simulink model "TB24_StageA_ModuleFault"  (R2025a)
settings: Solver=FixedStepDiscrete  StartTime=0  StopTime=TB.t_end  FixedStep=TB.dt  RelTol=1e-3
InitFcn:
  | % 모델과 같은 폴더의 초기화 스크립트를 실행해 P(설계 파라미터)와 TB(시험 조건)를 만든다.
  | run(fullfile(fileparts(get_param(bdroot, 'FileName')), 'TB24_init.m'));
values from neighbouring files (symbols this model uses):
  TB = struct()    [TB24_init.m]    (also in run_TB24.m = evalin('base', 'TB'))
libraries: fl_lib x126, nesl_utility x55
(part 2 of 3)

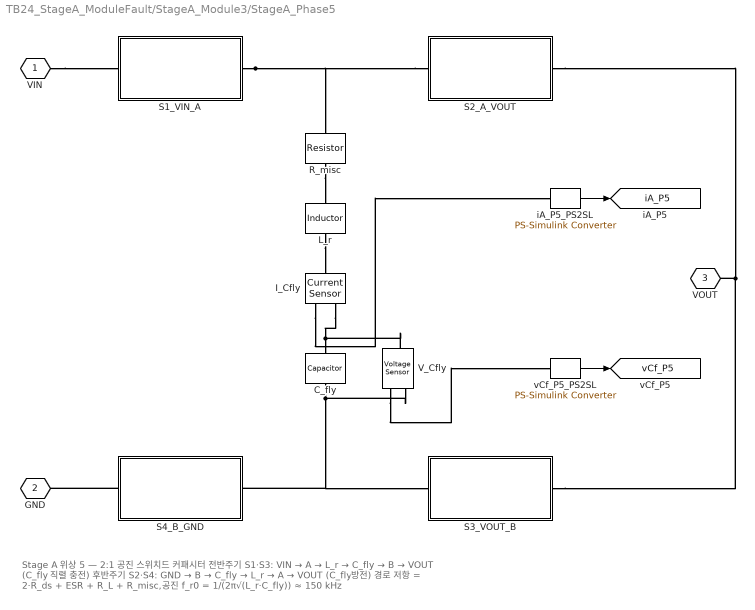
== system TB24_StageA_ModuleFault/StageA_Module3/StageA_Phase5 ==
  note: Stage A 위상 5 — 2:1 공진 스위치드 커패시터
      | 전반주기 S1·S3: VIN → A → L_r → C_fly → B → VOUT (C_fly 직렬 충전)
      | 후반주기 S2·S4: GND → B → C_fly → L_r → A → VOUT (C_fly 방전)
      | 경로 저항 = 2·R_ds + ESR + R_L + R_misc, 공진 f_r0 = 1/(2π√(L_r·C_fly)) ≈ 150 kHz
  C_fly : fl_lib/Electrical/Electrical Elements/Capacitor  c=TB.A.Cfly F  r=TB.A.ESR Ohm  g=0 1/Ohm  i_specify=off  i_priority=None  i=0 A  i_nominal_specify=off  i_nominal_value=1  i_nominal_unit=A  v_specify=off  v_priority=None  v=0 V  v_nominal_specify=off  v_nominal_value=1  v_nominal_unit=V  vc_specify=on  vc_priority=High  vc=TB.vC0_ph(5) V  vc_nominal_specify=off  vc_nominal_value=1  vc_nominal_unit=V
  I_Cfly : fl_lib/Electrical/Electrical Sensors/Current Sensor
  L_r : fl_lib/Electrical/Electrical Elements/Inductor  l=TB.A.Lr H  r=TB.A.RL Ohm  g=1e-9 1/Ohm  i_specify=off  i_priority=None  i=0 A  i_nominal_specify=off  i_nominal_value=1  i_nominal_unit=A  v_specify=off  v_priority=None  v=0 V  v_nominal_specify=off  v_nominal_value=1  v_nominal_unit=V  i_L_specify=on  i_L_priority=High  i_L=0 A  i_L_nominal_specify=off  i_L_nominal_value=1  i_L_nominal_unit=A
  R_misc : fl_lib/Electrical/Electrical Elements/Resistor  R=TB.A.Rmisc Ohm  i_specify=off  i_priority=None  i=0 A  i_nominal_specify=off  i_nominal_value=1  i_nominal_unit=A  v_specify=off  v_priority=None  v=0 V  v_nominal_specify=off  v_nominal_value=1  v_nominal_unit=V
  S1_VIN_A : Subsystem  mask(PRISM-Hub switch cell){Ron=TB.A.Rds, Goff=TB.A.Goff, Vf=TB.A.Vf, Rd=TB.A.Rd, Goffd=TB.A.Goffd}
      mask prompts: Ron "도통 저항 R_on [Ohm]"; Goff "차단 컨덕턴스 G_off [S]"; Vf "다이오드 순방향 전압 Vf [V]"; Rd "다이오드 도통 저항 R_d [Ohm]"; Goffd "다이오드 차단 컨덕턴스 [S]"
      mask help: 전력 반도체 스위치 셀 S1. 게이트 태그 gA_P5_S1.
      settings: AttributesFormatString=gate: gA_P5_S1
      mask Display:
      | plot([0.05 0.35 ],[0.50 0.50 ],[0.35 0.65 ],[0.50 0.74 ],[0.65 0.95 ],[0.50 0.50 ]);
      | plot([0.20 0.20 0.42 ],[0.50 0.20 0.20 ],[0.58 0.80 0.80 ],[0.20 0.20 0.50 ]);
      | plot([0.42 0.58 0.58 0.42 ],[0.20 0.10 0.30 0.20 ],[0.42 0.42 ],[0.10 0.30 ]);
      | text(0.5,0.80,'S1','horizontalAlignment','center','texmode','off');
      | port_label('LConn',1,'D');
      | port_label('RConn',1,'S');
  S2_A_VOUT : Subsystem  mask(PRISM-Hub switch cell){Ron=TB.A.Rds, Goff=TB.A.Goff, Vf=TB.A.Vf, Rd=TB.A.Rd, Goffd=TB.A.Goffd}
      mask prompts: Ron "도통 저항 R_on [Ohm]"; Goff "차단 컨덕턴스 G_off [S]"; Vf "다이오드 순방향 전압 Vf [V]"; Rd "다이오드 도통 저항 R_d [Ohm]"; Goffd "다이오드 차단 컨덕턴스 [S]"
      mask help: 전력 반도체 스위치 셀 S2. 게이트 태그 gA_P5_S2.
      settings: AttributesFormatString=gate: gA_P5_S2
      mask Display:
      | plot([0.05 0.35 ],[0.50 0.50 ],[0.35 0.65 ],[0.50 0.74 ],[0.65 0.95 ],[0.50 0.50 ]);
      | plot([0.20 0.20 0.42 ],[0.50 0.20 0.20 ],[0.58 0.80 0.80 ],[0.20 0.20 0.50 ]);
      | plot([0.42 0.58 0.58 0.42 ],[0.20 0.10 0.30 0.20 ],[0.42 0.42 ],[0.10 0.30 ]);
      | text(0.5,0.80,'S2','horizontalAlignment','center','texmode','off');
      | port_label('LConn',1,'D');
      | port_label('RConn',1,'S');
  S3_VOUT_B : Subsystem  mask(PRISM-Hub switch cell){Ron=TB.A.Rds, Goff=TB.A.Goff, Vf=TB.A.Vf, Rd=TB.A.Rd, Goffd=TB.A.Goffd}
      mask prompts: Ron "도통 저항 R_on [Ohm]"; Goff "차단 컨덕턴스 G_off [S]"; Vf "다이오드 순방향 전압 Vf [V]"; Rd "다이오드 도통 저항 R_d [Ohm]"; Goffd "다이오드 차단 컨덕턴스 [S]"
      mask help: 전력 반도체 스위치 셀 S3. 게이트 태그 gA_P5_S3.
      settings: AttributesFormatString=gate: gA_P5_S3
      mask Display:
      | plot([0.95 0.65 ],[0.50 0.50 ],[0.65 0.35 ],[0.50 0.74 ],[0.35 0.05 ],[0.50 0.50 ]);
      | plot([0.80 0.80 0.58 ],[0.50 0.20 0.20 ],[0.42 0.20 0.20 ],[0.20 0.20 0.50 ]);
      | plot([0.58 0.42 0.42 0.58 ],[0.20 0.10 0.30 0.20 ],[0.58 0.58 ],[0.10 0.30 ]);
      | text(0.5,0.80,'S3','horizontalAlignment','center','texmode','off');
      | port_label('LConn',1,'D');
      | port_label('RConn',1,'S');
  S4_B_GND : Subsystem  mask(PRISM-Hub switch cell){Ron=TB.A.Rds, Goff=TB.A.Goff, Vf=TB.A.Vf, Rd=TB.A.Rd, Goffd=TB.A.Goffd}
      mask prompts: Ron "도통 저항 R_on [Ohm]"; Goff "차단 컨덕턴스 G_off [S]"; Vf "다이오드 순방향 전압 Vf [V]"; Rd "다이오드 도통 저항 R_d [Ohm]"; Goffd "다이오드 차단 컨덕턴스 [S]"
      mask help: 전력 반도체 스위치 셀 S4. 게이트 태그 gA_P5_S4.
      settings: AttributesFormatString=gate: gA_P5_S4
      mask Display:
      | plot([0.95 0.65 ],[0.50 0.50 ],[0.65 0.35 ],[0.50 0.74 ],[0.35 0.05 ],[0.50 0.50 ]);
      | plot([0.80 0.80 0.58 ],[0.50 0.20 0.20 ],[0.42 0.20 0.20 ],[0.20 0.20 0.50 ]);
      | plot([0.58 0.42 0.42 0.58 ],[0.20 0.10 0.30 0.20 ],[0.58 0.58 ],[0.10 0.30 ]);
      | text(0.5,0.80,'S4','horizontalAlignment','center','texmode','off');
      | port_label('LConn',1,'D');
      | port_label('RConn',1,'S');
  V_Cfly : fl_lib/Electrical/Electrical Sensors/Voltage Sensor
  iA_P5_PS2SL : nesl_utility/PS-Simulink Converter  PhysicalDomain=network_engine_domain  SubClassName=ps_output  LeftPortType=input  RightPortType=output  PseudoPeriodic=off  Frequencies=[]  VectorFormat=inherit  Unit=inherit  AffineConversion=off
  vCf_P5_PS2SL : nesl_utility/PS-Simulink Converter  PhysicalDomain=network_engine_domain  SubClassName=ps_output  LeftPortType=input  RightPortType=output  PseudoPeriodic=off  Frequencies=[]  VectorFormat=inherit  Unit=inherit  AffineConversion=off
  VIN : PMIOPort  Side=Left
  GND : PMIOPort  Port=2  Side=Left
  VOUT : PMIOPort  Port=3  Side=Right
  tag scope: iA_P5=global, vCf_P5=global
  wires:
  iA_P5_PS2SL/1 -> [iA_P5]
  vCf_P5_PS2SL/1 -> [vCf_P5]
  connections:
  VIN/RConn1 -- S1_VIN_A/LConn1
  S2_A_VOUT/LConn1 -- S1_VIN_A/RConn1 -- R_misc/LConn1
  R_misc/RConn1 -- L_r/LConn1
  L_r/RConn1 -- I_Cfly/LConn1
  C_fly/LConn1 -- I_Cfly/RConn2 -- V_Cfly/LConn1
  S4_B_GND/LConn1 -- C_fly/RConn1 -- S3_VOUT_B/RConn1 -- V_Cfly/RConn2
  S4_B_GND/RConn1 -- GND/RConn1
  VOUT/RConn1 -- S2_A_VOUT/RConn1 -- S3_VOUT_B/LConn1
  I_Cfly/RConn1 -- iA_P5_PS2SL/LConn1
  V_Cfly/RConn1 -- vCf_P5_PS2SL/LConn1

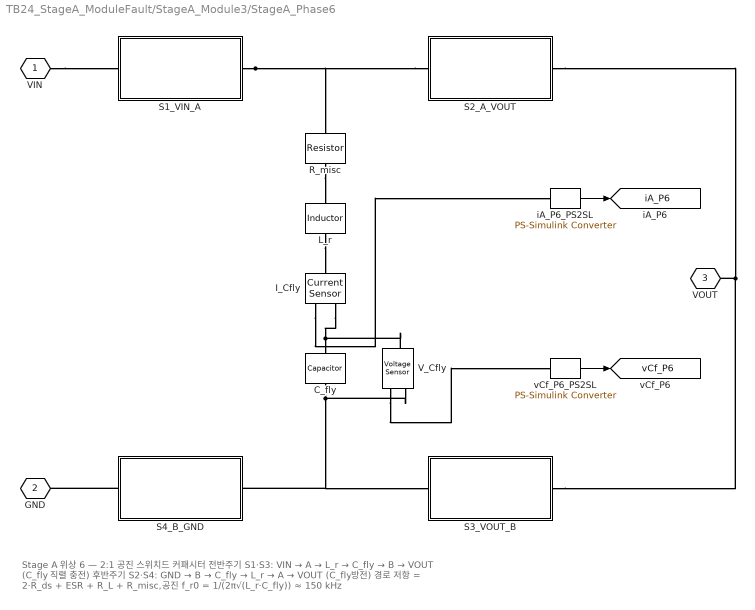
== system TB24_StageA_ModuleFault/StageA_Module3/StageA_Phase6 ==
  note: Stage A 위상 6 — 2:1 공진 스위치드 커패시터
      | 전반주기 S1·S3: VIN → A → L_r → C_fly → B → VOUT (C_fly 직렬 충전)
      | 후반주기 S2·S4: GND → B → C_fly → L_r → A → VOUT (C_fly 방전)
      | 경로 저항 = 2·R_ds + ESR + R_L + R_misc, 공진 f_r0 = 1/(2π√(L_r·C_fly)) ≈ 150 kHz
  C_fly : fl_lib/Electrical/Electrical Elements/Capacitor  c=TB.A.Cfly F  r=TB.A.ESR Ohm  g=0 1/Ohm  i_specify=off  i_priority=None  i=0 A  i_nominal_specify=off  i_nominal_value=1  i_nominal_unit=A  v_specify=off  v_priority=None  v=0 V  v_nominal_specify=off  v_nominal_value=1  v_nominal_unit=V  vc_specify=on  vc_priority=High  vc=TB.vC0_ph(6) V  vc_nominal_specify=off  vc_nominal_value=1  vc_nominal_unit=V
  I_Cfly : fl_lib/Electrical/Electrical Sensors/Current Sensor
  L_r : fl_lib/Electrical/Electrical Elements/Inductor  l=TB.A.Lr H  r=TB.A.RL Ohm  g=1e-9 1/Ohm  i_specify=off  i_priority=None  i=0 A  i_nominal_specify=off  i_nominal_value=1  i_nominal_unit=A  v_specify=off  v_priority=None  v=0 V  v_nominal_specify=off  v_nominal_value=1  v_nominal_unit=V  i_L_specify=on  i_L_priority=High  i_L=0 A  i_L_nominal_specify=off  i_L_nominal_value=1  i_L_nominal_unit=A
  R_misc : fl_lib/Electrical/Electrical Elements/Resistor  R=TB.A.Rmisc Ohm  i_specify=off  i_priority=None  i=0 A  i_nominal_specify=off  i_nominal_value=1  i_nominal_unit=A  v_specify=off  v_priority=None  v=0 V  v_nominal_specify=off  v_nominal_value=1  v_nominal_unit=V
  S1_VIN_A : Subsystem  mask(PRISM-Hub switch cell){Ron=TB.A.Rds, Goff=TB.A.Goff, Vf=TB.A.Vf, Rd=TB.A.Rd, Goffd=TB.A.Goffd}
      mask prompts: Ron "도통 저항 R_on [Ohm]"; Goff "차단 컨덕턴스 G_off [S]"; Vf "다이오드 순방향 전압 Vf [V]"; Rd "다이오드 도통 저항 R_d [Ohm]"; Goffd "다이오드 차단 컨덕턴스 [S]"
      mask help: 전력 반도체 스위치 셀 S1. 게이트 태그 gA_P6_S1.
      settings: AttributesFormatString=gate: gA_P6_S1
      mask Display:
      | plot([0.05 0.35 ],[0.50 0.50 ],[0.35 0.65 ],[0.50 0.74 ],[0.65 0.95 ],[0.50 0.50 ]);
      | plot([0.20 0.20 0.42 ],[0.50 0.20 0.20 ],[0.58 0.80 0.80 ],[0.20 0.20 0.50 ]);
      | plot([0.42 0.58 0.58 0.42 ],[0.20 0.10 0.30 0.20 ],[0.42 0.42 ],[0.10 0.30 ]);
      | text(0.5,0.80,'S1','horizontalAlignment','center','texmode','off');
      | port_label('LConn',1,'D');
      | port_label('RConn',1,'S');
  S2_A_VOUT : Subsystem  mask(PRISM-Hub switch cell){Ron=TB.A.Rds, Goff=TB.A.Goff, Vf=TB.A.Vf, Rd=TB.A.Rd, Goffd=TB.A.Goffd}
      mask prompts: Ron "도통 저항 R_on [Ohm]"; Goff "차단 컨덕턴스 G_off [S]"; Vf "다이오드 순방향 전압 Vf [V]"; Rd "다이오드 도통 저항 R_d [Ohm]"; Goffd "다이오드 차단 컨덕턴스 [S]"
      mask help: 전력 반도체 스위치 셀 S2. 게이트 태그 gA_P6_S2.
      settings: AttributesFormatString=gate: gA_P6_S2
      mask Display:
      | plot([0.05 0.35 ],[0.50 0.50 ],[0.35 0.65 ],[0.50 0.74 ],[0.65 0.95 ],[0.50 0.50 ]);
      | plot([0.20 0.20 0.42 ],[0.50 0.20 0.20 ],[0.58 0.80 0.80 ],[0.20 0.20 0.50 ]);
      | plot([0.42 0.58 0.58 0.42 ],[0.20 0.10 0.30 0.20 ],[0.42 0.42 ],[0.10 0.30 ]);
      | text(0.5,0.80,'S2','horizontalAlignment','center','texmode','off');
      | port_label('LConn',1,'D');
      | port_label('RConn',1,'S');
  S3_VOUT_B : Subsystem  mask(PRISM-Hub switch cell){Ron=TB.A.Rds, Goff=TB.A.Goff, Vf=TB.A.Vf, Rd=TB.A.Rd, Goffd=TB.A.Goffd}
      mask prompts: Ron "도통 저항 R_on [Ohm]"; Goff "차단 컨덕턴스 G_off [S]"; Vf "다이오드 순방향 전압 Vf [V]"; Rd "다이오드 도통 저항 R_d [Ohm]"; Goffd "다이오드 차단 컨덕턴스 [S]"
      mask help: 전력 반도체 스위치 셀 S3. 게이트 태그 gA_P6_S3.
      settings: AttributesFormatString=gate: gA_P6_S3
      mask Display:
      | plot([0.95 0.65 ],[0.50 0.50 ],[0.65 0.35 ],[0.50 0.74 ],[0.35 0.05 ],[0.50 0.50 ]);
      | plot([0.80 0.80 0.58 ],[0.50 0.20 0.20 ],[0.42 0.20 0.20 ],[0.20 0.20 0.50 ]);
      | plot([0.58 0.42 0.42 0.58 ],[0.20 0.10 0.30 0.20 ],[0.58 0.58 ],[0.10 0.30 ]);
      | text(0.5,0.80,'S3','horizontalAlignment','center','texmode','off');
      | port_label('LConn',1,'D');
      | port_label('RConn',1,'S');
  S4_B_GND : Subsystem  mask(PRISM-Hub switch cell){Ron=TB.A.Rds, Goff=TB.A.Goff, Vf=TB.A.Vf, Rd=TB.A.Rd, Goffd=TB.A.Goffd}
      mask prompts: Ron "도통 저항 R_on [Ohm]"; Goff "차단 컨덕턴스 G_off [S]"; Vf "다이오드 순방향 전압 Vf [V]"; Rd "다이오드 도통 저항 R_d [Ohm]"; Goffd "다이오드 차단 컨덕턴스 [S]"
      mask help: 전력 반도체 스위치 셀 S4. 게이트 태그 gA_P6_S4.
      settings: AttributesFormatString=gate: gA_P6_S4
      mask Display:
      | plot([0.95 0.65 ],[0.50 0.50 ],[0.65 0.35 ],[0.50 0.74 ],[0.35 0.05 ],[0.50 0.50 ]);
      | plot([0.80 0.80 0.58 ],[0.50 0.20 0.20 ],[0.42 0.20 0.20 ],[0.20 0.20 0.50 ]);
      | plot([0.58 0.42 0.42 0.58 ],[0.20 0.10 0.30 0.20 ],[0.58 0.58 ],[0.10 0.30 ]);
      | text(0.5,0.80,'S4','horizontalAlignment','center','texmode','off');
      | port_label('LConn',1,'D');
      | port_label('RConn',1,'S');
  V_Cfly : fl_lib/Electrical/Electrical Sensors/Voltage Sensor
  iA_P6_PS2SL : nesl_utility/PS-Simulink Converter  PhysicalDomain=network_engine_domain  SubClassName=ps_output  LeftPortType=input  RightPortType=output  PseudoPeriodic=off  Frequencies=[]  VectorFormat=inherit  Unit=inherit  AffineConversion=off
  vCf_P6_PS2SL : nesl_utility/PS-Simulink Converter  PhysicalDomain=network_engine_domain  SubClassName=ps_output  LeftPortType=input  RightPortType=output  PseudoPeriodic=off  Frequencies=[]  VectorFormat=inherit  Unit=inherit  AffineConversion=off
  VIN : PMIOPort  Side=Left
  GND : PMIOPort  Port=2  Side=Left
  VOUT : PMIOPort  Port=3  Side=Right
  tag scope: iA_P6=global, vCf_P6=global
  wires:
  iA_P6_PS2SL/1 -> [iA_P6]
  vCf_P6_PS2SL/1 -> [vCf_P6]
  connections:
  VIN/RConn1 -- S1_VIN_A/LConn1
  S2_A_VOUT/LConn1 -- S1_VIN_A/RConn1 -- R_misc/LConn1
  R_misc/RConn1 -- L_r/LConn1
  L_r/RConn1 -- I_Cfly/LConn1
  C_fly/LConn1 -- I_Cfly/RConn2 -- V_Cfly/LConn1
  S4_B_GND/LConn1 -- C_fly/RConn1 -- S3_VOUT_B/RConn1 -- V_Cfly/RConn2
  S4_B_GND/RConn1 -- GND/RConn1
  VOUT/RConn1 -- S2_A_VOUT/RConn1 -- S3_VOUT_B/LConn1
  I_Cfly/RConn1 -- iA_P6_PS2SL/LConn1
  V_Cfly/RConn1 -- vCf_P6_PS2SL/LConn1

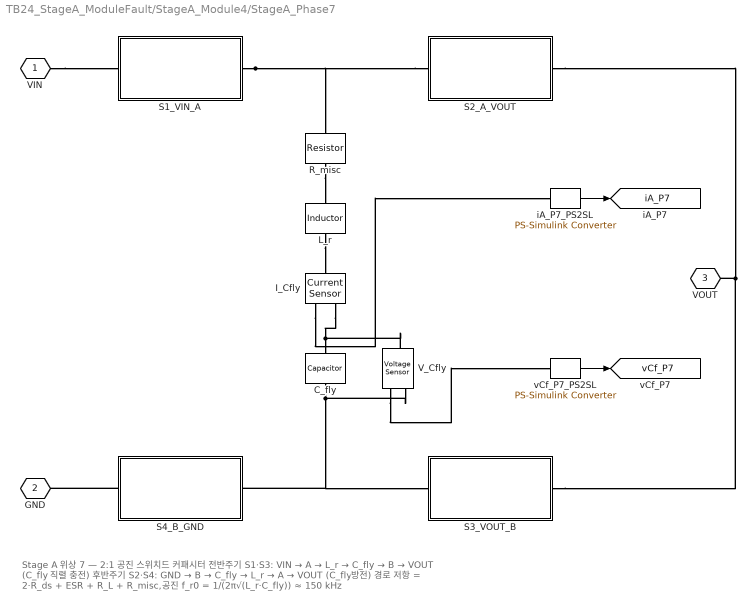
== system TB24_StageA_ModuleFault/StageA_Module4/StageA_Phase7 ==
  note: Stage A 위상 7 — 2:1 공진 스위치드 커패시터
      | 전반주기 S1·S3: VIN → A → L_r → C_fly → B → VOUT (C_fly 직렬 충전)
      | 후반주기 S2·S4: GND → B → C_fly → L_r → A → VOUT (C_fly 방전)
      | 경로 저항 = 2·R_ds + ESR + R_L + R_misc, 공진 f_r0 = 1/(2π√(L_r·C_fly)) ≈ 150 kHz
  C_fly : fl_lib/Electrical/Electrical Elements/Capacitor  c=TB.A.Cfly F  r=TB.A.ESR Ohm  g=0 1/Ohm  i_specify=off  i_priority=None  i=0 A  i_nominal_specify=off  i_nominal_value=1  i_nominal_unit=A  v_specify=off  v_priority=None  v=0 V  v_nominal_specify=off  v_nominal_value=1  v_nominal_unit=V  vc_specify=on  vc_priority=High  vc=TB.vC0_ph(7) V  vc_nominal_specify=off  vc_nominal_value=1  vc_nominal_unit=V
  I_Cfly : fl_lib/Electrical/Electrical Sensors/Current Sensor
  L_r : fl_lib/Electrical/Electrical Elements/Inductor  l=TB.A.Lr H  r=TB.A.RL Ohm  g=1e-9 1/Ohm  i_specify=off  i_priority=None  i=0 A  i_nominal_specify=off  i_nominal_value=1  i_nominal_unit=A  v_specify=off  v_priority=None  v=0 V  v_nominal_specify=off  v_nominal_value=1  v_nominal_unit=V  i_L_specify=on  i_L_priority=High  i_L=0 A  i_L_nominal_specify=off  i_L_nominal_value=1  i_L_nominal_unit=A
  R_misc : fl_lib/Electrical/Electrical Elements/Resistor  R=TB.A.Rmisc Ohm  i_specify=off  i_priority=None  i=0 A  i_nominal_specify=off  i_nominal_value=1  i_nominal_unit=A  v_specify=off  v_priority=None  v=0 V  v_nominal_specify=off  v_nominal_value=1  v_nominal_unit=V
  S1_VIN_A : Subsystem  mask(PRISM-Hub switch cell){Ron=TB.A.Rds, Goff=TB.A.Goff, Vf=TB.A.Vf, Rd=TB.A.Rd, Goffd=TB.A.Goffd}
      mask prompts: Ron "도통 저항 R_on [Ohm]"; Goff "차단 컨덕턴스 G_off [S]"; Vf "다이오드 순방향 전압 Vf [V]"; Rd "다이오드 도통 저항 R_d [Ohm]"; Goffd "다이오드 차단 컨덕턴스 [S]"
      mask help: 전력 반도체 스위치 셀 S1. 게이트 태그 gA_P7_S1.
      settings: AttributesFormatString=gate: gA_P7_S1
      mask Display:
      | plot([0.05 0.35 ],[0.50 0.50 ],[0.35 0.65 ],[0.50 0.74 ],[0.65 0.95 ],[0.50 0.50 ]);
      | plot([0.20 0.20 0.42 ],[0.50 0.20 0.20 ],[0.58 0.80 0.80 ],[0.20 0.20 0.50 ]);
      | plot([0.42 0.58 0.58 0.42 ],[0.20 0.10 0.30 0.20 ],[0.42 0.42 ],[0.10 0.30 ]);
      | text(0.5,0.80,'S1','horizontalAlignment','center','texmode','off');
      | port_label('LConn',1,'D');
      | port_label('RConn',1,'S');
  S2_A_VOUT : Subsystem  mask(PRISM-Hub switch cell){Ron=TB.A.Rds, Goff=TB.A.Goff, Vf=TB.A.Vf, Rd=TB.A.Rd, Goffd=TB.A.Goffd}
      mask prompts: Ron "도통 저항 R_on [Ohm]"; Goff "차단 컨덕턴스 G_off [S]"; Vf "다이오드 순방향 전압 Vf [V]"; Rd "다이오드 도통 저항 R_d [Ohm]"; Goffd "다이오드 차단 컨덕턴스 [S]"
      mask help: 전력 반도체 스위치 셀 S2. 게이트 태그 gA_P7_S2.
      settings: AttributesFormatString=gate: gA_P7_S2
      mask Display:
      | plot([0.05 0.35 ],[0.50 0.50 ],[0.35 0.65 ],[0.50 0.74 ],[0.65 0.95 ],[0.50 0.50 ]);
      | plot([0.20 0.20 0.42 ],[0.50 0.20 0.20 ],[0.58 0.80 0.80 ],[0.20 0.20 0.50 ]);
      | plot([0.42 0.58 0.58 0.42 ],[0.20 0.10 0.30 0.20 ],[0.42 0.42 ],[0.10 0.30 ]);
      | text(0.5,0.80,'S2','horizontalAlignment','center','texmode','off');
      | port_label('LConn',1,'D');
      | port_label('RConn',1,'S');
  S3_VOUT_B : Subsystem  mask(PRISM-Hub switch cell){Ron=TB.A.Rds, Goff=TB.A.Goff, Vf=TB.A.Vf, Rd=TB.A.Rd, Goffd=TB.A.Goffd}
      mask prompts: Ron "도통 저항 R_on [Ohm]"; Goff "차단 컨덕턴스 G_off [S]"; Vf "다이오드 순방향 전압 Vf [V]"; Rd "다이오드 도통 저항 R_d [Ohm]"; Goffd "다이오드 차단 컨덕턴스 [S]"
      mask help: 전력 반도체 스위치 셀 S3. 게이트 태그 gA_P7_S3.
      settings: AttributesFormatString=gate: gA_P7_S3
      mask Display:
      | plot([0.95 0.65 ],[0.50 0.50 ],[0.65 0.35 ],[0.50 0.74 ],[0.35 0.05 ],[0.50 0.50 ]);
      | plot([0.80 0.80 0.58 ],[0.50 0.20 0.20 ],[0.42 0.20 0.20 ],[0.20 0.20 0.50 ]);
      | plot([0.58 0.42 0.42 0.58 ],[0.20 0.10 0.30 0.20 ],[0.58 0.58 ],[0.10 0.30 ]);
      | text(0.5,0.80,'S3','horizontalAlignment','center','texmode','off');
      | port_label('LConn',1,'D');
      | port_label('RConn',1,'S');
  S4_B_GND : Subsystem  mask(PRISM-Hub switch cell){Ron=TB.A.Rds, Goff=TB.A.Goff, Vf=TB.A.Vf, Rd=TB.A.Rd, Goffd=TB.A.Goffd}
      mask prompts: Ron "도통 저항 R_on [Ohm]"; Goff "차단 컨덕턴스 G_off [S]"; Vf "다이오드 순방향 전압 Vf [V]"; Rd "다이오드 도통 저항 R_d [Ohm]"; Goffd "다이오드 차단 컨덕턴스 [S]"
      mask help: 전력 반도체 스위치 셀 S4. 게이트 태그 gA_P7_S4.
      settings: AttributesFormatString=gate: gA_P7_S4
      mask Display:
      | plot([0.95 0.65 ],[0.50 0.50 ],[0.65 0.35 ],[0.50 0.74 ],[0.35 0.05 ],[0.50 0.50 ]);
      | plot([0.80 0.80 0.58 ],[0.50 0.20 0.20 ],[0.42 0.20 0.20 ],[0.20 0.20 0.50 ]);
      | plot([0.58 0.42 0.42 0.58 ],[0.20 0.10 0.30 0.20 ],[0.58 0.58 ],[0.10 0.30 ]);
      | text(0.5,0.80,'S4','horizontalAlignment','center','texmode','off');
      | port_label('LConn',1,'D');
      | port_label('RConn',1,'S');
  V_Cfly : fl_lib/Electrical/Electrical Sensors/Voltage Sensor
  iA_P7_PS2SL : nesl_utility/PS-Simulink Converter  PhysicalDomain=network_engine_domain  SubClassName=ps_output  LeftPortType=input  RightPortType=output  PseudoPeriodic=off  Frequencies=[]  VectorFormat=inherit  Unit=inherit  AffineConversion=off
  vCf_P7_PS2SL : nesl_utility/PS-Simulink Converter  PhysicalDomain=network_engine_domain  SubClassName=ps_output  LeftPortType=input  RightPortType=output  PseudoPeriodic=off  Frequencies=[]  VectorFormat=inherit  Unit=inherit  AffineConversion=off
  VIN : PMIOPort  Side=Left
  GND : PMIOPort  Port=2  Side=Left
  VOUT : PMIOPort  Port=3  Side=Right
  tag scope: iA_P7=global, vCf_P7=global
  wires:
  iA_P7_PS2SL/1 -> [iA_P7]
  vCf_P7_PS2SL/1 -> [vCf_P7]
  connections:
  VIN/RConn1 -- S1_VIN_A/LConn1
  S2_A_VOUT/LConn1 -- S1_VIN_A/RConn1 -- R_misc/LConn1
  R_misc/RConn1 -- L_r/LConn1
  L_r/RConn1 -- I_Cfly/LConn1
  C_fly/LConn1 -- I_Cfly/RConn2 -- V_Cfly/LConn1
  S4_B_GND/LConn1 -- C_fly/RConn1 -- S3_VOUT_B/RConn1 -- V_Cfly/RConn2
  S4_B_GND/RConn1 -- GND/RConn1
  VOUT/RConn1 -- S2_A_VOUT/RConn1 -- S3_VOUT_B/LConn1
  I_Cfly/RConn1 -- iA_P7_PS2SL/LConn1
  V_Cfly/RConn1 -- vCf_P7_PS2SL/LConn1

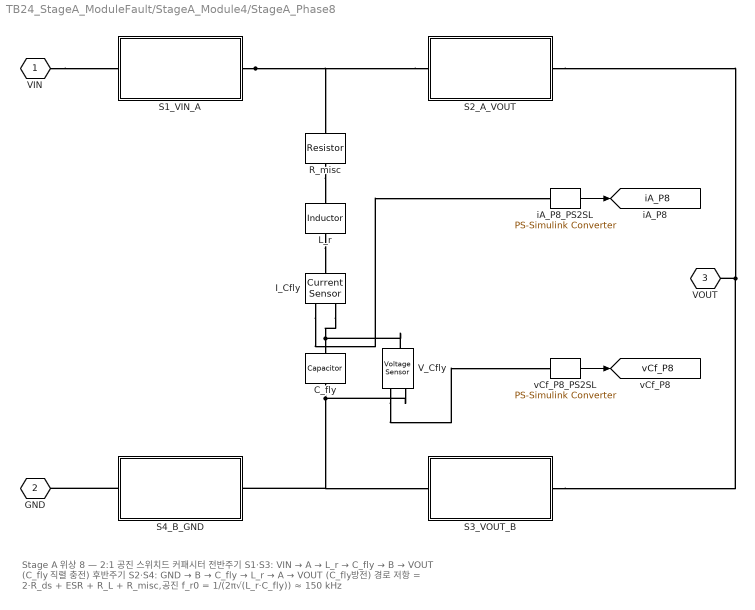
== system TB24_StageA_ModuleFault/StageA_Module4/StageA_Phase8 ==
  note: Stage A 위상 8 — 2:1 공진 스위치드 커패시터
      | 전반주기 S1·S3: VIN → A → L_r → C_fly → B → VOUT (C_fly 직렬 충전)
      | 후반주기 S2·S4: GND → B → C_fly → L_r → A → VOUT (C_fly 방전)
      | 경로 저항 = 2·R_ds + ESR + R_L + R_misc, 공진 f_r0 = 1/(2π√(L_r·C_fly)) ≈ 150 kHz
  C_fly : fl_lib/Electrical/Electrical Elements/Capacitor  c=TB.A.Cfly F  r=TB.A.ESR Ohm  g=0 1/Ohm  i_specify=off  i_priority=None  i=0 A  i_nominal_specify=off  i_nominal_value=1  i_nominal_unit=A  v_specify=off  v_priority=None  v=0 V  v_nominal_specify=off  v_nominal_value=1  v_nominal_unit=V  vc_specify=on  vc_priority=High  vc=TB.vC0_ph(8) V  vc_nominal_specify=off  vc_nominal_value=1  vc_nominal_unit=V
  I_Cfly : fl_lib/Electrical/Electrical Sensors/Current Sensor
  L_r : fl_lib/Electrical/Electrical Elements/Inductor  l=TB.A.Lr H  r=TB.A.RL Ohm  g=1e-9 1/Ohm  i_specify=off  i_priority=None  i=0 A  i_nominal_specify=off  i_nominal_value=1  i_nominal_unit=A  v_specify=off  v_priority=None  v=0 V  v_nominal_specify=off  v_nominal_value=1  v_nominal_unit=V  i_L_specify=on  i_L_priority=High  i_L=0 A  i_L_nominal_specify=off  i_L_nominal_value=1  i_L_nominal_unit=A
  R_misc : fl_lib/Electrical/Electrical Elements/Resistor  R=TB.A.Rmisc Ohm  i_specify=off  i_priority=None  i=0 A  i_nominal_specify=off  i_nominal_value=1  i_nominal_unit=A  v_specify=off  v_priority=None  v=0 V  v_nominal_specify=off  v_nominal_value=1  v_nominal_unit=V
  S1_VIN_A : Subsystem  mask(PRISM-Hub switch cell){Ron=TB.A.Rds, Goff=TB.A.Goff, Vf=TB.A.Vf, Rd=TB.A.Rd, Goffd=TB.A.Goffd}
      mask prompts: Ron "도통 저항 R_on [Ohm]"; Goff "차단 컨덕턴스 G_off [S]"; Vf "다이오드 순방향 전압 Vf [V]"; Rd "다이오드 도통 저항 R_d [Ohm]"; Goffd "다이오드 차단 컨덕턴스 [S]"
      mask help: 전력 반도체 스위치 셀 S1. 게이트 태그 gA_P8_S1.
      settings: AttributesFormatString=gate: gA_P8_S1
      mask Display:
      | plot([0.05 0.35 ],[0.50 0.50 ],[0.35 0.65 ],[0.50 0.74 ],[0.65 0.95 ],[0.50 0.50 ]);
      | plot([0.20 0.20 0.42 ],[0.50 0.20 0.20 ],[0.58 0.80 0.80 ],[0.20 0.20 0.50 ]);
      | plot([0.42 0.58 0.58 0.42 ],[0.20 0.10 0.30 0.20 ],[0.42 0.42 ],[0.10 0.30 ]);
      | text(0.5,0.80,'S1','horizontalAlignment','center','texmode','off');
      | port_label('LConn',1,'D');
      | port_label('RConn',1,'S');
  S2_A_VOUT : Subsystem  mask(PRISM-Hub switch cell){Ron=TB.A.Rds, Goff=TB.A.Goff, Vf=TB.A.Vf, Rd=TB.A.Rd, Goffd=TB.A.Goffd}
      mask prompts: Ron "도통 저항 R_on [Ohm]"; Goff "차단 컨덕턴스 G_off [S]"; Vf "다이오드 순방향 전압 Vf [V]"; Rd "다이오드 도통 저항 R_d [Ohm]"; Goffd "다이오드 차단 컨덕턴스 [S]"
      mask help: 전력 반도체 스위치 셀 S2. 게이트 태그 gA_P8_S2.
      settings: AttributesFormatString=gate: gA_P8_S2
      mask Display:
      | plot([0.05 0.35 ],[0.50 0.50 ],[0.35 0.65 ],[0.50 0.74 ],[0.65 0.95 ],[0.50 0.50 ]);
      | plot([0.20 0.20 0.42 ],[0.50 0.20 0.20 ],[0.58 0.80 0.80 ],[0.20 0.20 0.50 ]);
      | plot([0.42 0.58 0.58 0.42 ],[0.20 0.10 0.30 0.20 ],[0.42 0.42 ],[0.10 0.30 ]);
      | text(0.5,0.80,'S2','horizontalAlignment','center','texmode','off');
      | port_label('LConn',1,'D');
      | port_label('RConn',1,'S');
  S3_VOUT_B : Subsystem  mask(PRISM-Hub switch cell){Ron=TB.A.Rds, Goff=TB.A.Goff, Vf=TB.A.Vf, Rd=TB.A.Rd, Goffd=TB.A.Goffd}
      mask prompts: Ron "도통 저항 R_on [Ohm]"; Goff "차단 컨덕턴스 G_off [S]"; Vf "다이오드 순방향 전압 Vf [V]"; Rd "다이오드 도통 저항 R_d [Ohm]"; Goffd "다이오드 차단 컨덕턴스 [S]"
      mask help: 전력 반도체 스위치 셀 S3. 게이트 태그 gA_P8_S3.
      settings: AttributesFormatString=gate: gA_P8_S3
      mask Display:
      | plot([0.95 0.65 ],[0.50 0.50 ],[0.65 0.35 ],[0.50 0.74 ],[0.35 0.05 ],[0.50 0.50 ]);
      | plot([0.80 0.80 0.58 ],[0.50 0.20 0.20 ],[0.42 0.20 0.20 ],[0.20 0.20 0.50 ]);
      | plot([0.58 0.42 0.42 0.58 ],[0.20 0.10 0.30 0.20 ],[0.58 0.58 ],[0.10 0.30 ]);
      | text(0.5,0.80,'S3','horizontalAlignment','center','texmode','off');
      | port_label('LConn',1,'D');
      | port_label('RConn',1,'S');
  S4_B_GND : Subsystem  mask(PRISM-Hub switch cell){Ron=TB.A.Rds, Goff=TB.A.Goff, Vf=TB.A.Vf, Rd=TB.A.Rd, Goffd=TB.A.Goffd}
      mask prompts: Ron "도통 저항 R_on [Ohm]"; Goff "차단 컨덕턴스 G_off [S]"; Vf "다이오드 순방향 전압 Vf [V]"; Rd "다이오드 도통 저항 R_d [Ohm]"; Goffd "다이오드 차단 컨덕턴스 [S]"
      mask help: 전력 반도체 스위치 셀 S4. 게이트 태그 gA_P8_S4.
      settings: AttributesFormatString=gate: gA_P8_S4
      mask Display:
      | plot([0.95 0.65 ],[0.50 0.50 ],[0.65 0.35 ],[0.50 0.74 ],[0.35 0.05 ],[0.50 0.50 ]);
      | plot([0.80 0.80 0.58 ],[0.50 0.20 0.20 ],[0.42 0.20 0.20 ],[0.20 0.20 0.50 ]);
      | plot([0.58 0.42 0.42 0.58 ],[0.20 0.10 0.30 0.20 ],[0.58 0.58 ],[0.10 0.30 ]);
      | text(0.5,0.80,'S4','horizontalAlignment','center','texmode','off');
      | port_label('LConn',1,'D');
      | port_label('RConn',1,'S');
  V_Cfly : fl_lib/Electrical/Electrical Sensors/Voltage Sensor
  iA_P8_PS2SL : nesl_utility/PS-Simulink Converter  PhysicalDomain=network_engine_domain  SubClassName=ps_output  LeftPortType=input  RightPortType=output  PseudoPeriodic=off  Frequencies=[]  VectorFormat=inherit  Unit=inherit  AffineConversion=off
  vCf_P8_PS2SL : nesl_utility/PS-Simulink Converter  PhysicalDomain=network_engine_domain  SubClassName=ps_output  LeftPortType=input  RightPortType=output  PseudoPeriodic=off  Frequencies=[]  VectorFormat=inherit  Unit=inherit  AffineConversion=off
  VIN : PMIOPort  Side=Left
  GND : PMIOPort  Port=2  Side=Left
  VOUT : PMIOPort  Port=3  Side=Right
  tag scope: iA_P8=global, vCf_P8=global
  wires:
  iA_P8_PS2SL/1 -> [iA_P8]
  vCf_P8_PS2SL/1 -> [vCf_P8]
  connections:
  VIN/RConn1 -- S1_VIN_A/LConn1
  S2_A_VOUT/LConn1 -- S1_VIN_A/RConn1 -- R_misc/LConn1
  R_misc/RConn1 -- L_r/LConn1
  L_r/RConn1 -- I_Cfly/LConn1
  C_fly/LConn1 -- I_Cfly/RConn2 -- V_Cfly/LConn1
  S4_B_GND/LConn1 -- C_fly/RConn1 -- S3_VOUT_B/RConn1 -- V_Cfly/RConn2
  S4_B_GND/RConn1 -- GND/RConn1
  VOUT/RConn1 -- S2_A_VOUT/RConn1 -- S3_VOUT_B/LConn1
  I_Cfly/RConn1 -- iA_P8_PS2SL/LConn1
  V_Cfly/RConn1 -- vCf_P8_PS2SL/LConn1

== system TB24_StageA_ModuleFault/StageA_Module1/StageA_Phase1/S1_VIN_A ==
  note: 스위치 셀: 이상 스위치(R_on, G_off) + 역병렬 바디 다이오드(Vf, R_d)
      | 게이트: 전역 태그 "gA_P1_S1" (> 0.5 이면 도통)
  D_body : fl_lib/Electrical/Electrical Elements/Diode  Vf=Vf V  Ron=Rd Ohm  Goff=Goffd 1/Ohm  i_specify=off  i_priority=None  i=0 A  i_nominal_specify=off  i_nominal_value=1  i_nominal_unit=A  v_specify=off  v_priority=None  v=0 V  v_nominal_specify=off  v_nominal_value=1  v_nominal_unit=V
  Gate_PS : nesl_utility/Simulink-PS Converter  PhysicalDomain=network_engine_domain  SubClassName=ps_input  LeftPortType=input  RightPortType=output  PseudoPeriodic=off  Frequencies=[]  NoiseDistribution=none  NoiseParameters=[]  Unit=1  AffineConversion=off  FilteringAndDerivatives=zero  SimscapeFilterOrder=1  InputFilterTimeConstant=0.001  UdotUserProvided=0
  SW : fl_lib/Electrical/Electrical Elements/Switch  R_closed=Ron Ohm  G_open=Goff 1/Ohm  Threshold=0.5  i_specify=off  i_priority=None  i=0 A  i_nominal_specify=off  i_nominal_value=1  i_nominal_unit=A  v_specify=off  v_priority=None  v=0 V  v_nominal_specify=off  v_nominal_value=1  v_nominal_unit=V
  D : PMIOPort  Side=Left
  S : PMIOPort  Port=2  Side=Right
  wires:
  [gA_P1_S1] -> Gate_PS/1
  connections:
  Gate_PS/RConn1 -- SW/RConn1
  SW/LConn1 -- D/RConn1 -- D_body/RConn1
  S/RConn1 -- SW/RConn2 -- D_body/LConn1

== system TB24_StageA_ModuleFault/StageA_Module1/StageA_Phase1/S2_A_VOUT ==
  note: 스위치 셀: 이상 스위치(R_on, G_off) + 역병렬 바디 다이오드(Vf, R_d)
      | 게이트: 전역 태그 "gA_P1_S2" (> 0.5 이면 도통)
  D_body : fl_lib/Electrical/Electrical Elements/Diode  Vf=Vf V  Ron=Rd Ohm  Goff=Goffd 1/Ohm  i_specify=off  i_priority=None  i=0 A  i_nominal_specify=off  i_nominal_value=1  i_nominal_unit=A  v_specify=off  v_priority=None  v=0 V  v_nominal_specify=off  v_nominal_value=1  v_nominal_unit=V
  Gate_PS : nesl_utility/Simulink-PS Converter  PhysicalDomain=network_engine_domain  SubClassName=ps_input  LeftPortType=input  RightPortType=output  PseudoPeriodic=off  Frequencies=[]  NoiseDistribution=none  NoiseParameters=[]  Unit=1  AffineConversion=off  FilteringAndDerivatives=zero  SimscapeFilterOrder=1  InputFilterTimeConstant=0.001  UdotUserProvided=0
  SW : fl_lib/Electrical/Electrical Elements/Switch  R_closed=Ron Ohm  G_open=Goff 1/Ohm  Threshold=0.5  i_specify=off  i_priority=None  i=0 A  i_nominal_specify=off  i_nominal_value=1  i_nominal_unit=A  v_specify=off  v_priority=None  v=0 V  v_nominal_specify=off  v_nominal_value=1  v_nominal_unit=V
  D : PMIOPort  Side=Left
  S : PMIOPort  Port=2  Side=Right
  wires:
  [gA_P1_S2] -> Gate_PS/1
  connections:
  Gate_PS/RConn1 -- SW/RConn1
  SW/LConn1 -- D/RConn1 -- D_body/RConn1
  S/RConn1 -- SW/RConn2 -- D_body/LConn1

== system TB24_StageA_ModuleFault/StageA_Module1/StageA_Phase1/S3_VOUT_B ==
  note: 스위치 셀: 이상 스위치(R_on, G_off) + 역병렬 바디 다이오드(Vf, R_d)
      | 게이트: 전역 태그 "gA_P1_S3" (> 0.5 이면 도통)
  D_body : fl_lib/Electrical/Electrical Elements/Diode  Vf=Vf V  Ron=Rd Ohm  Goff=Goffd 1/Ohm  i_specify=off  i_priority=None  i=0 A  i_nominal_specify=off  i_nominal_value=1  i_nominal_unit=A  v_specify=off  v_priority=None  v=0 V  v_nominal_specify=off  v_nominal_value=1  v_nominal_unit=V
  Gate_PS : nesl_utility/Simulink-PS Converter  PhysicalDomain=network_engine_domain  SubClassName=ps_input  LeftPortType=input  RightPortType=output  PseudoPeriodic=off  Frequencies=[]  NoiseDistribution=none  NoiseParameters=[]  Unit=1  AffineConversion=off  FilteringAndDerivatives=zero  SimscapeFilterOrder=1  InputFilterTimeConstant=0.001  UdotUserProvided=0
  SW : fl_lib/Electrical/Electrical Elements/Switch  R_closed=Ron Ohm  G_open=Goff 1/Ohm  Threshold=0.5  i_specify=off  i_priority=None  i=0 A  i_nominal_specify=off  i_nominal_value=1  i_nominal_unit=A  v_specify=off  v_priority=None  v=0 V  v_nominal_specify=off  v_nominal_value=1  v_nominal_unit=V
  D : PMIOPort  Side=Left
  S : PMIOPort  Port=2  Side=Right
  wires:
  [gA_P1_S3] -> Gate_PS/1
  connections:
  Gate_PS/RConn1 -- SW/RConn1
  SW/LConn1 -- D/RConn1 -- D_body/RConn1
  S/RConn1 -- SW/RConn2 -- D_body/LConn1

== system TB24_StageA_ModuleFault/StageA_Module1/StageA_Phase1/S4_B_GND ==
  note: 스위치 셀: 이상 스위치(R_on, G_off) + 역병렬 바디 다이오드(Vf, R_d)
      | 게이트: 전역 태그 "gA_P1_S4" (> 0.5 이면 도통)
  D_body : fl_lib/Electrical/Electrical Elements/Diode  Vf=Vf V  Ron=Rd Ohm  Goff=Goffd 1/Ohm  i_specify=off  i_priority=None  i=0 A  i_nominal_specify=off  i_nominal_value=1  i_nominal_unit=A  v_specify=off  v_priority=None  v=0 V  v_nominal_specify=off  v_nominal_value=1  v_nominal_unit=V
  Gate_PS : nesl_utility/Simulink-PS Converter  PhysicalDomain=network_engine_domain  SubClassName=ps_input  LeftPortType=input  RightPortType=output  PseudoPeriodic=off  Frequencies=[]  NoiseDistribution=none  NoiseParameters=[]  Unit=1  AffineConversion=off  FilteringAndDerivatives=zero  SimscapeFilterOrder=1  InputFilterTimeConstant=0.001  UdotUserProvided=0
  SW : fl_lib/Electrical/Electrical Elements/Switch  R_closed=Ron Ohm  G_open=Goff 1/Ohm  Threshold=0.5  i_specify=off  i_priority=None  i=0 A  i_nominal_specify=off  i_nominal_value=1  i_nominal_unit=A  v_specify=off  v_priority=None  v=0 V  v_nominal_specify=off  v_nominal_value=1  v_nominal_unit=V
  D : PMIOPort  Side=Left
  S : PMIOPort  Port=2  Side=Right
  wires:
  [gA_P1_S4] -> Gate_PS/1
  connections:
  Gate_PS/RConn1 -- SW/RConn1
  SW/LConn1 -- D/RConn1 -- D_body/RConn1
  S/RConn1 -- SW/RConn2 -- D_body/LConn1

== system TB24_StageA_ModuleFault/StageA_Module1/StageA_Phase2/S1_VIN_A ==
  note: 스위치 셀: 이상 스위치(R_on, G_off) + 역병렬 바디 다이오드(Vf, R_d)
      | 게이트: 전역 태그 "gA_P2_S1" (> 0.5 이면 도통)
  D_body : fl_lib/Electrical/Electrical Elements/Diode  Vf=Vf V  Ron=Rd Ohm  Goff=Goffd 1/Ohm  i_specify=off  i_priority=None  i=0 A  i_nominal_specify=off  i_nominal_value=1  i_nominal_unit=A  v_specify=off  v_priority=None  v=0 V  v_nominal_specify=off  v_nominal_value=1  v_nominal_unit=V
  Gate_PS : nesl_utility/Simulink-PS Converter  PhysicalDomain=network_engine_domain  SubClassName=ps_input  LeftPortType=input  RightPortType=output  PseudoPeriodic=off  Frequencies=[]  NoiseDistribution=none  NoiseParameters=[]  Unit=1  AffineConversion=off  FilteringAndDerivatives=zero  SimscapeFilterOrder=1  InputFilterTimeConstant=0.001  UdotUserProvided=0
  SW : fl_lib/Electrical/Electrical Elements/Switch  R_closed=Ron Ohm  G_open=Goff 1/Ohm  Threshold=0.5  i_specify=off  i_priority=None  i=0 A  i_nominal_specify=off  i_nominal_value=1  i_nominal_unit=A  v_specify=off  v_priority=None  v=0 V  v_nominal_specify=off  v_nominal_value=1  v_nominal_unit=V
  D : PMIOPort  Side=Left
  S : PMIOPort  Port=2  Side=Right
  wires:
  [gA_P2_S1] -> Gate_PS/1
  connections:
  Gate_PS/RConn1 -- SW/RConn1
  SW/LConn1 -- D/RConn1 -- D_body/RConn1
  S/RConn1 -- SW/RConn2 -- D_body/LConn1

== system TB24_StageA_ModuleFault/StageA_Module1/StageA_Phase2/S2_A_VOUT ==
  note: 스위치 셀: 이상 스위치(R_on, G_off) + 역병렬 바디 다이오드(Vf, R_d)
      | 게이트: 전역 태그 "gA_P2_S2" (> 0.5 이면 도통)
  D_body : fl_lib/Electrical/Electrical Elements/Diode  Vf=Vf V  Ron=Rd Ohm  Goff=Goffd 1/Ohm  i_specify=off  i_priority=None  i=0 A  i_nominal_specify=off  i_nominal_value=1  i_nominal_unit=A  v_specify=off  v_priority=None  v=0 V  v_nominal_specify=off  v_nominal_value=1  v_nominal_unit=V
  Gate_PS : nesl_utility/Simulink-PS Converter  PhysicalDomain=network_engine_domain  SubClassName=ps_input  LeftPortType=input  RightPortType=output  PseudoPeriodic=off  Frequencies=[]  NoiseDistribution=none  NoiseParameters=[]  Unit=1  AffineConversion=off  FilteringAndDerivatives=zero  SimscapeFilterOrder=1  InputFilterTimeConstant=0.001  UdotUserProvided=0
  SW : fl_lib/Electrical/Electrical Elements/Switch  R_closed=Ron Ohm  G_open=Goff 1/Ohm  Threshold=0.5  i_specify=off  i_priority=None  i=0 A  i_nominal_specify=off  i_nominal_value=1  i_nominal_unit=A  v_specify=off  v_priority=None  v=0 V  v_nominal_specify=off  v_nominal_value=1  v_nominal_unit=V
  D : PMIOPort  Side=Left
  S : PMIOPort  Port=2  Side=Right
  wires:
  [gA_P2_S2] -> Gate_PS/1
  connections:
  Gate_PS/RConn1 -- SW/RConn1
  SW/LConn1 -- D/RConn1 -- D_body/RConn1
  S/RConn1 -- SW/RConn2 -- D_body/LConn1

== system TB24_StageA_ModuleFault/StageA_Module1/StageA_Phase2/S3_VOUT_B ==
  note: 스위치 셀: 이상 스위치(R_on, G_off) + 역병렬 바디 다이오드(Vf, R_d)
      | 게이트: 전역 태그 "gA_P2_S3" (> 0.5 이면 도통)
  D_body : fl_lib/Electrical/Electrical Elements/Diode  Vf=Vf V  Ron=Rd Ohm  Goff=Goffd 1/Ohm  i_specify=off  i_priority=None  i=0 A  i_nominal_specify=off  i_nominal_value=1  i_nominal_unit=A  v_specify=off  v_priority=None  v=0 V  v_nominal_specify=off  v_nominal_value=1  v_nominal_unit=V
  Gate_PS : nesl_utility/Simulink-PS Converter  PhysicalDomain=network_engine_domain  SubClassName=ps_input  LeftPortType=input  RightPortType=output  PseudoPeriodic=off  Frequencies=[]  NoiseDistribution=none  NoiseParameters=[]  Unit=1  AffineConversion=off  FilteringAndDerivatives=zero  SimscapeFilterOrder=1  InputFilterTimeConstant=0.001  UdotUserProvided=0
  SW : fl_lib/Electrical/Electrical Elements/Switch  R_closed=Ron Ohm  G_open=Goff 1/Ohm  Threshold=0.5  i_specify=off  i_priority=None  i=0 A  i_nominal_specify=off  i_nominal_value=1  i_nominal_unit=A  v_specify=off  v_priority=None  v=0 V  v_nominal_specify=off  v_nominal_value=1  v_nominal_unit=V
  D : PMIOPort  Side=Left
  S : PMIOPort  Port=2  Side=Right
  wires:
  [gA_P2_S3] -> Gate_PS/1
  connections:
  Gate_PS/RConn1 -- SW/RConn1
  SW/LConn1 -- D/RConn1 -- D_body/RConn1
  S/RConn1 -- SW/RConn2 -- D_body/LConn1

== system TB24_StageA_ModuleFault/StageA_Module1/StageA_Phase2/S4_B_GND ==
  note: 스위치 셀: 이상 스위치(R_on, G_off) + 역병렬 바디 다이오드(Vf, R_d)
      | 게이트: 전역 태그 "gA_P2_S4" (> 0.5 이면 도통)
  D_body : fl_lib/Electrical/Electrical Elements/Diode  Vf=Vf V  Ron=Rd Ohm  Goff=Goffd 1/Ohm  i_specify=off  i_priority=None  i=0 A  i_nominal_specify=off  i_nominal_value=1  i_nominal_unit=A  v_specify=off  v_priority=None  v=0 V  v_nominal_specify=off  v_nominal_value=1  v_nominal_unit=V
  Gate_PS : nesl_utility/Simulink-PS Converter  PhysicalDomain=network_engine_domain  SubClassName=ps_input  LeftPortType=input  RightPortType=output  PseudoPeriodic=off  Frequencies=[]  NoiseDistribution=none  NoiseParameters=[]  Unit=1  AffineConversion=off  FilteringAndDerivatives=zero  SimscapeFilterOrder=1  InputFilterTimeConstant=0.001  UdotUserProvided=0
  SW : fl_lib/Electrical/Electrical Elements/Switch  R_closed=Ron Ohm  G_open=Goff 1/Ohm  Threshold=0.5  i_specify=off  i_priority=None  i=0 A  i_nominal_specify=off  i_nominal_value=1  i_nominal_unit=A  v_specify=off  v_priority=None  v=0 V  v_nominal_specify=off  v_nominal_value=1  v_nominal_unit=V
  D : PMIOPort  Side=Left
  S : PMIOPort  Port=2  Side=Right
  wires:
  [gA_P2_S4] -> Gate_PS/1
  connections:
  Gate_PS/RConn1 -- SW/RConn1
  SW/LConn1 -- D/RConn1 -- D_body/RConn1
  S/RConn1 -- SW/RConn2 -- D_body/LConn1

== system TB24_StageA_ModuleFault/StageA_Module2/StageA_Phase3/S1_VIN_A ==
  note: 스위치 셀: 이상 스위치(R_on, G_off) + 역병렬 바디 다이오드(Vf, R_d)
      | 게이트: 전역 태그 "gA_P3_S1" (> 0.5 이면 도통)
  D_body : fl_lib/Electrical/Electrical Elements/Diode  Vf=Vf V  Ron=Rd Ohm  Goff=Goffd 1/Ohm  i_specify=off  i_priority=None  i=0 A  i_nominal_specify=off  i_nominal_value=1  i_nominal_unit=A  v_specify=off  v_priority=None  v=0 V  v_nominal_specify=off  v_nominal_value=1  v_nominal_unit=V
  Gate_PS : nesl_utility/Simulink-PS Converter  PhysicalDomain=network_engine_domain  SubClassName=ps_input  LeftPortType=input  RightPortType=output  PseudoPeriodic=off  Frequencies=[]  NoiseDistribution=none  NoiseParameters=[]  Unit=1  AffineConversion=off  FilteringAndDerivatives=zero  SimscapeFilterOrder=1  InputFilterTimeConstant=0.001  UdotUserProvided=0
  SW : fl_lib/Electrical/Electrical Elements/Switch  R_closed=Ron Ohm  G_open=Goff 1/Ohm  Threshold=0.5  i_specify=off  i_priority=None  i=0 A  i_nominal_specify=off  i_nominal_value=1  i_nominal_unit=A  v_specify=off  v_priority=None  v=0 V  v_nominal_specify=off  v_nominal_value=1  v_nominal_unit=V
  D : PMIOPort  Side=Left
  S : PMIOPort  Port=2  Side=Right
  wires:
  [gA_P3_S1] -> Gate_PS/1
  connections:
  Gate_PS/RConn1 -- SW/RConn1
  SW/LConn1 -- D/RConn1 -- D_body/RConn1
  S/RConn1 -- SW/RConn2 -- D_body/LConn1

== system TB24_StageA_ModuleFault/StageA_Module2/StageA_Phase3/S2_A_VOUT ==
  note: 스위치 셀: 이상 스위치(R_on, G_off) + 역병렬 바디 다이오드(Vf, R_d)
      | 게이트: 전역 태그 "gA_P3_S2" (> 0.5 이면 도통)
  D_body : fl_lib/Electrical/Electrical Elements/Diode  Vf=Vf V  Ron=Rd Ohm  Goff=Goffd 1/Ohm  i_specify=off  i_priority=None  i=0 A  i_nominal_specify=off  i_nominal_value=1  i_nominal_unit=A  v_specify=off  v_priority=None  v=0 V  v_nominal_specify=off  v_nominal_value=1  v_nominal_unit=V
  Gate_PS : nesl_utility/Simulink-PS Converter  PhysicalDomain=network_engine_domain  SubClassName=ps_input  LeftPortType=input  RightPortType=output  PseudoPeriodic=off  Frequencies=[]  NoiseDistribution=none  NoiseParameters=[]  Unit=1  AffineConversion=off  FilteringAndDerivatives=zero  SimscapeFilterOrder=1  InputFilterTimeConstant=0.001  UdotUserProvided=0
  SW : fl_lib/Electrical/Electrical Elements/Switch  R_closed=Ron Ohm  G_open=Goff 1/Ohm  Threshold=0.5  i_specify=off  i_priority=None  i=0 A  i_nominal_specify=off  i_nominal_value=1  i_nominal_unit=A  v_specify=off  v_priority=None  v=0 V  v_nominal_specify=off  v_nominal_value=1  v_nominal_unit=V
  D : PMIOPort  Side=Left
  S : PMIOPort  Port=2  Side=Right
  wires:
  [gA_P3_S2] -> Gate_PS/1
  connections:
  Gate_PS/RConn1 -- SW/RConn1
  SW/LConn1 -- D/RConn1 -- D_body/RConn1
  S/RConn1 -- SW/RConn2 -- D_body/LConn1

== system TB24_StageA_ModuleFault/StageA_Module2/StageA_Phase3/S3_VOUT_B ==
  note: 스위치 셀: 이상 스위치(R_on, G_off) + 역병렬 바디 다이오드(Vf, R_d)
      | 게이트: 전역 태그 "gA_P3_S3" (> 0.5 이면 도통)
  D_body : fl_lib/Electrical/Electrical Elements/Diode  Vf=Vf V  Ron=Rd Ohm  Goff=Goffd 1/Ohm  i_specify=off  i_priority=None  i=0 A  i_nominal_specify=off  i_nominal_value=1  i_nominal_unit=A  v_specify=off  v_priority=None  v=0 V  v_nominal_specify=off  v_nominal_value=1  v_nominal_unit=V
  Gate_PS : nesl_utility/Simulink-PS Converter  PhysicalDomain=network_engine_domain  SubClassName=ps_input  LeftPortType=input  RightPortType=output  PseudoPeriodic=off  Frequencies=[]  NoiseDistribution=none  NoiseParameters=[]  Unit=1  AffineConversion=off  FilteringAndDerivatives=zero  SimscapeFilterOrder=1  InputFilterTimeConstant=0.001  UdotUserProvided=0
  SW : fl_lib/Electrical/Electrical Elements/Switch  R_closed=Ron Ohm  G_open=Goff 1/Ohm  Threshold=0.5  i_specify=off  i_priority=None  i=0 A  i_nominal_specify=off  i_nominal_value=1  i_nominal_unit=A  v_specify=off  v_priority=None  v=0 V  v_nominal_specify=off  v_nominal_value=1  v_nominal_unit=V
  D : PMIOPort  Side=Left
  S : PMIOPort  Port=2  Side=Right
  wires:
  [gA_P3_S3] -> Gate_PS/1
  connections:
  Gate_PS/RConn1 -- SW/RConn1
  SW/LConn1 -- D/RConn1 -- D_body/RConn1
  S/RConn1 -- SW/RConn2 -- D_body/LConn1

== system TB24_StageA_ModuleFault/StageA_Module2/StageA_Phase3/S4_B_GND ==
  note: 스위치 셀: 이상 스위치(R_on, G_off) + 역병렬 바디 다이오드(Vf, R_d)
      | 게이트: 전역 태그 "gA_P3_S4" (> 0.5 이면 도통)
  D_body : fl_lib/Electrical/Electrical Elements/Diode  Vf=Vf V  Ron=Rd Ohm  Goff=Goffd 1/Ohm  i_specify=off  i_priority=None  i=0 A  i_nominal_specify=off  i_nominal_value=1  i_nominal_unit=A  v_specify=off  v_priority=None  v=0 V  v_nominal_specify=off  v_nominal_value=1  v_nominal_unit=V
  Gate_PS : nesl_utility/Simulink-PS Converter  PhysicalDomain=network_engine_domain  SubClassName=ps_input  LeftPortType=input  RightPortType=output  PseudoPeriodic=off  Frequencies=[]  NoiseDistribution=none  NoiseParameters=[]  Unit=1  AffineConversion=off  FilteringAndDerivatives=zero  SimscapeFilterOrder=1  InputFilterTimeConstant=0.001  UdotUserProvided=0
  SW : fl_lib/Electrical/Electrical Elements/Switch  R_closed=Ron Ohm  G_open=Goff 1/Ohm  Threshold=0.5  i_specify=off  i_priority=None  i=0 A  i_nominal_specify=off  i_nominal_value=1  i_nominal_unit=A  v_specify=off  v_priority=None  v=0 V  v_nominal_specify=off  v_nominal_value=1  v_nominal_unit=V
  D : PMIOPort  Side=Left
  S : PMIOPort  Port=2  Side=Right
  wires:
  [gA_P3_S4] -> Gate_PS/1
  connections:
  Gate_PS/RConn1 -- SW/RConn1
  SW/LConn1 -- D/RConn1 -- D_body/RConn1
  S/RConn1 -- SW/RConn2 -- D_body/LConn1

== system TB24_StageA_ModuleFault/StageA_Module2/StageA_Phase4/S1_VIN_A ==
  note: 스위치 셀: 이상 스위치(R_on, G_off) + 역병렬 바디 다이오드(Vf, R_d)
      | 게이트: 전역 태그 "gA_P4_S1" (> 0.5 이면 도통)
  D_body : fl_lib/Electrical/Electrical Elements/Diode  Vf=Vf V  Ron=Rd Ohm  Goff=Goffd 1/Ohm  i_specify=off  i_priority=None  i=0 A  i_nominal_specify=off  i_nominal_value=1  i_nominal_unit=A  v_specify=off  v_priority=None  v=0 V  v_nominal_specify=off  v_nominal_value=1  v_nominal_unit=V
  Gate_PS : nesl_utility/Simulink-PS Converter  PhysicalDomain=network_engine_domain  SubClassName=ps_input  LeftPortType=input  RightPortType=output  PseudoPeriodic=off  Frequencies=[]  NoiseDistribution=none  NoiseParameters=[]  Unit=1  AffineConversion=off  FilteringAndDerivatives=zero  SimscapeFilterOrder=1  InputFilterTimeConstant=0.001  UdotUserProvided=0
  SW : fl_lib/Electrical/Electrical Elements/Switch  R_closed=Ron Ohm  G_open=Goff 1/Ohm  Threshold=0.5  i_specify=off  i_priority=None  i=0 A  i_nominal_specify=off  i_nominal_value=1  i_nominal_unit=A  v_specify=off  v_priority=None  v=0 V  v_nominal_specify=off  v_nominal_value=1  v_nominal_unit=V
  D : PMIOPort  Side=Left
  S : PMIOPort  Port=2  Side=Right
  wires:
  [gA_P4_S1] -> Gate_PS/1
  connections:
  Gate_PS/RConn1 -- SW/RConn1
  SW/LConn1 -- D/RConn1 -- D_body/RConn1
  S/RConn1 -- SW/RConn2 -- D_body/LConn1

== system TB24_StageA_ModuleFault/StageA_Module2/StageA_Phase4/S2_A_VOUT ==
  note: 스위치 셀: 이상 스위치(R_on, G_off) + 역병렬 바디 다이오드(Vf, R_d)
      | 게이트: 전역 태그 "gA_P4_S2" (> 0.5 이면 도통)
  D_body : fl_lib/Electrical/Electrical Elements/Diode  Vf=Vf V  Ron=Rd Ohm  Goff=Goffd 1/Ohm  i_specify=off  i_priority=None  i=0 A  i_nominal_specify=off  i_nominal_value=1  i_nominal_unit=A  v_specify=off  v_priority=None  v=0 V  v_nominal_specify=off  v_nominal_value=1  v_nominal_unit=V
  Gate_PS : nesl_utility/Simulink-PS Converter  PhysicalDomain=network_engine_domain  SubClassName=ps_input  LeftPortType=input  RightPortType=output  PseudoPeriodic=off  Frequencies=[]  NoiseDistribution=none  NoiseParameters=[]  Unit=1  AffineConversion=off  FilteringAndDerivatives=zero  SimscapeFilterOrder=1  InputFilterTimeConstant=0.001  UdotUserProvided=0
  SW : fl_lib/Electrical/Electrical Elements/Switch  R_closed=Ron Ohm  G_open=Goff 1/Ohm  Threshold=0.5  i_specify=off  i_priority=None  i=0 A  i_nominal_specify=off  i_nominal_value=1  i_nominal_unit=A  v_specify=off  v_priority=None  v=0 V  v_nominal_specify=off  v_nominal_value=1  v_nominal_unit=V
  D : PMIOPort  Side=Left
  S : PMIOPort  Port=2  Side=Right
  wires:
  [gA_P4_S2] -> Gate_PS/1
  connections:
  Gate_PS/RConn1 -- SW/RConn1
  SW/LConn1 -- D/RConn1 -- D_body/RConn1
  S/RConn1 -- SW/RConn2 -- D_body/LConn1

== system TB24_StageA_ModuleFault/StageA_Module2/StageA_Phase4/S3_VOUT_B ==
  note: 스위치 셀: 이상 스위치(R_on, G_off) + 역병렬 바디 다이오드(Vf, R_d)
      | 게이트: 전역 태그 "gA_P4_S3" (> 0.5 이면 도통)
  D_body : fl_lib/Electrical/Electrical Elements/Diode  Vf=Vf V  Ron=Rd Ohm  Goff=Goffd 1/Ohm  i_specify=off  i_priority=None  i=0 A  i_nominal_specify=off  i_nominal_value=1  i_nominal_unit=A  v_specify=off  v_priority=None  v=0 V  v_nominal_specify=off  v_nominal_value=1  v_nominal_unit=V
  Gate_PS : nesl_utility/Simulink-PS Converter  PhysicalDomain=network_engine_domain  SubClassName=ps_input  LeftPortType=input  RightPortType=output  PseudoPeriodic=off  Frequencies=[]  NoiseDistribution=none  NoiseParameters=[]  Unit=1  AffineConversion=off  FilteringAndDerivatives=zero  SimscapeFilterOrder=1  InputFilterTimeConstant=0.001  UdotUserProvided=0
  SW : fl_lib/Electrical/Electrical Elements/Switch  R_closed=Ron Ohm  G_open=Goff 1/Ohm  Threshold=0.5  i_specify=off  i_priority=None  i=0 A  i_nominal_specify=off  i_nominal_value=1  i_nominal_unit=A  v_specify=off  v_priority=None  v=0 V  v_nominal_specify=off  v_nominal_value=1  v_nominal_unit=V
  D : PMIOPort  Side=Left
  S : PMIOPort  Port=2  Side=Right
  wires:
  [gA_P4_S3] -> Gate_PS/1
  connections:
  Gate_PS/RConn1 -- SW/RConn1
  SW/LConn1 -- D/RConn1 -- D_body/RConn1
  S/RConn1 -- SW/RConn2 -- D_body/LConn1

== system TB24_StageA_ModuleFault/StageA_Module2/StageA_Phase4/S4_B_GND ==
  note: 스위치 셀: 이상 스위치(R_on, G_off) + 역병렬 바디 다이오드(Vf, R_d)
      | 게이트: 전역 태그 "gA_P4_S4" (> 0.5 이면 도통)
  D_body : fl_lib/Electrical/Electrical Elements/Diode  Vf=Vf V  Ron=Rd Ohm  Goff=Goffd 1/Ohm  i_specify=off  i_priority=None  i=0 A  i_nominal_specify=off  i_nominal_value=1  i_nominal_unit=A  v_specify=off  v_priority=None  v=0 V  v_nominal_specify=off  v_nominal_value=1  v_nominal_unit=V
  Gate_PS : nesl_utility/Simulink-PS Converter  PhysicalDomain=network_engine_domain  SubClassName=ps_input  LeftPortType=input  RightPortType=output  PseudoPeriodic=off  Frequencies=[]  NoiseDistribution=none  NoiseParameters=[]  Unit=1  AffineConversion=off  FilteringAndDerivatives=zero  SimscapeFilterOrder=1  InputFilterTimeConstant=0.001  UdotUserProvided=0
  SW : fl_lib/Electrical/Electrical Elements/Switch  R_closed=Ron Ohm  G_open=Goff 1/Ohm  Threshold=0.5  i_specify=off  i_priority=None  i=0 A  i_nominal_specify=off  i_nominal_value=1  i_nominal_unit=A  v_specify=off  v_priority=None  v=0 V  v_nominal_specify=off  v_nominal_value=1  v_nominal_unit=V
  D : PMIOPort  Side=Left
  S : PMIOPort  Port=2  Side=Right
  wires:
  [gA_P4_S4] -> Gate_PS/1
  connections:
  Gate_PS/RConn1 -- SW/RConn1
  SW/LConn1 -- D/RConn1 -- D_body/RConn1
  S/RConn1 -- SW/RConn2 -- D_body/LConn1

== system TB24_StageA_ModuleFault/StageA_Module3/StageA_Phase5/S1_VIN_A ==
  note: 스위치 셀: 이상 스위치(R_on, G_off) + 역병렬 바디 다이오드(Vf, R_d)
      | 게이트: 전역 태그 "gA_P5_S1" (> 0.5 이면 도통)
  D_body : fl_lib/Electrical/Electrical Elements/Diode  Vf=Vf V  Ron=Rd Ohm  Goff=Goffd 1/Ohm  i_specify=off  i_priority=None  i=0 A  i_nominal_specify=off  i_nominal_value=1  i_nominal_unit=A  v_specify=off  v_priority=None  v=0 V  v_nominal_specify=off  v_nominal_value=1  v_nominal_unit=V
  Gate_PS : nesl_utility/Simulink-PS Converter  PhysicalDomain=network_engine_domain  SubClassName=ps_input  LeftPortType=input  RightPortType=output  PseudoPeriodic=off  Frequencies=[]  NoiseDistribution=none  NoiseParameters=[]  Unit=1  AffineConversion=off  FilteringAndDerivatives=zero  SimscapeFilterOrder=1  InputFilterTimeConstant=0.001  UdotUserProvided=0
  SW : fl_lib/Electrical/Electrical Elements/Switch  R_closed=Ron Ohm  G_open=Goff 1/Ohm  Threshold=0.5  i_specify=off  i_priority=None  i=0 A  i_nominal_specify=off  i_nominal_value=1  i_nominal_unit=A  v_specify=off  v_priority=None  v=0 V  v_nominal_specify=off  v_nominal_value=1  v_nominal_unit=V
  D : PMIOPort  Side=Left
  S : PMIOPort  Port=2  Side=Right
  wires:
  [gA_P5_S1] -> Gate_PS/1
  connections:
  Gate_PS/RConn1 -- SW/RConn1
  SW/LConn1 -- D/RConn1 -- D_body/RConn1
  S/RConn1 -- SW/RConn2 -- D_body/LConn1

== system TB24_StageA_ModuleFault/StageA_Module3/StageA_Phase5/S2_A_VOUT ==
  note: 스위치 셀: 이상 스위치(R_on, G_off) + 역병렬 바디 다이오드(Vf, R_d)
      | 게이트: 전역 태그 "gA_P5_S2" (> 0.5 이면 도통)
  D_body : fl_lib/Electrical/Electrical Elements/Diode  Vf=Vf V  Ron=Rd Ohm  Goff=Goffd 1/Ohm  i_specify=off  i_priority=None  i=0 A  i_nominal_specify=off  i_nominal_value=1  i_nominal_unit=A  v_specify=off  v_priority=None  v=0 V  v_nominal_specify=off  v_nominal_value=1  v_nominal_unit=V
  Gate_PS : nesl_utility/Simulink-PS Converter  PhysicalDomain=network_engine_domain  SubClassName=ps_input  LeftPortType=input  RightPortType=output  PseudoPeriodic=off  Frequencies=[]  NoiseDistribution=none  NoiseParameters=[]  Unit=1  AffineConversion=off  FilteringAndDerivatives=zero  SimscapeFilterOrder=1  InputFilterTimeConstant=0.001  UdotUserProvided=0
  SW : fl_lib/Electrical/Electrical Elements/Switch  R_closed=Ron Ohm  G_open=Goff 1/Ohm  Threshold=0.5  i_specify=off  i_priority=None  i=0 A  i_nominal_specify=off  i_nominal_value=1  i_nominal_unit=A  v_specify=off  v_priority=None  v=0 V  v_nominal_specify=off  v_nominal_value=1  v_nominal_unit=V
  D : PMIOPort  Side=Left
  S : PMIOPort  Port=2  Side=Right
  wires:
  [gA_P5_S2] -> Gate_PS/1
  connections:
  Gate_PS/RConn1 -- SW/RConn1
  SW/LConn1 -- D/RConn1 -- D_body/RConn1
  S/RConn1 -- SW/RConn2 -- D_body/LConn1

== system TB24_StageA_ModuleFault/StageA_Module3/StageA_Phase5/S3_VOUT_B ==
  note: 스위치 셀: 이상 스위치(R_on, G_off) + 역병렬 바디 다이오드(Vf, R_d)
      | 게이트: 전역 태그 "gA_P5_S3" (> 0.5 이면 도통)
  D_body : fl_lib/Electrical/Electrical Elements/Diode  Vf=Vf V  Ron=Rd Ohm  Goff=Goffd 1/Ohm  i_specify=off  i_priority=None  i=0 A  i_nominal_specify=off  i_nominal_value=1  i_nominal_unit=A  v_specify=off  v_priority=None  v=0 V  v_nominal_specify=off  v_nominal_value=1  v_nominal_unit=V
  Gate_PS : nesl_utility/Simulink-PS Converter  PhysicalDomain=network_engine_domain  SubClassName=ps_input  LeftPortType=input  RightPortType=output  PseudoPeriodic=off  Frequencies=[]  NoiseDistribution=none  NoiseParameters=[]  Unit=1  AffineConversion=off  FilteringAndDerivatives=zero  SimscapeFilterOrder=1  InputFilterTimeConstant=0.001  UdotUserProvided=0
  SW : fl_lib/Electrical/Electrical Elements/Switch  R_closed=Ron Ohm  G_open=Goff 1/Ohm  Threshold=0.5  i_specify=off  i_priority=None  i=0 A  i_nominal_specify=off  i_nominal_value=1  i_nominal_unit=A  v_specify=off  v_priority=None  v=0 V  v_nominal_specify=off  v_nominal_value=1  v_nominal_unit=V
  D : PMIOPort  Side=Left
  S : PMIOPort  Port=2  Side=Right
  wires:
  [gA_P5_S3] -> Gate_PS/1
  connections:
  Gate_PS/RConn1 -- SW/RConn1
  SW/LConn1 -- D/RConn1 -- D_body/RConn1
  S/RConn1 -- SW/RConn2 -- D_body/LConn1
